simulink model "nonlinear_closed_backstepping_0"  (R2023b)
settings: Solver=ode45  StartTime=0.0  StopTime=100  FixedStep=0.001  MaxStep=1e-3  RelTol=1e-3  EnableMultiTasking=on
PreLoadFcn:
  | S=load('rovmodel75kg.mat'); M_nom=S.M; Ma_nom=S.Ma; DL_nom=S.DL; clear S;
values from neighbouring files (symbols this model uses):
  B = 735.75    [rovmodel75kg.mat]
  DL = [3.221 0 0 0 0 0 0 3.291 0 0 0 0 ... (36 elements, 6x6)]    [rovmodel75kg.mat]
  DQ = [105.3 0 0 0 0 0 0 139.6 0 0 0 0 ... (36 elements, 6x6)]    [rovmodel75kg.mat]
  I = [2.51  0  0; 0  3.38  0.01; 0  0.01  1.73]    [rovmodel75kg.mat]
  m = [75  0  0; 0  75  0; 0  0  75]    [rovmodel75kg.mat]
  M = [75 0 0 0 0 0 0 75 0 0 0 0 ... (36 elements, 6x6)]    [rovmodel75kg.mat]
  Ma = [-20.392 0 0 0 0 0 0 -53.435 0 0 0 0 ... (36 elements, 6x6)]    [rovmodel75kg.mat]
  rg = [0 0 0]    [rovmodel75kg.mat]
  W = 735.75    [rovmodel75kg.mat]
  zb = -0.397    [rovmodel75kg.mat]
  zg = 0    [rovmodel75kg.mat]
libraries: matrix_library x6
settings Model: Creator=Joshua cheng  LastModifiedBy=yhm
settings SolverCC: AlgebraicLoopSolver=TrustRegion
settings DataIOCC: LimitDataPoints=on  SaveFormat=Array  SignalLoggingSaveFormat=ModelDataLogs  ReturnWorkspaceOutputs=off
settings OptimizationCC: BlockReduction=off  OptimizeBlockIOStorage=off  BufferReuse=off  GlobalBufferReuse=off  ExpressionFolding=off  ExpressionDepthLimit=2147483647  LocalBlockOutputs=off  LifeSpan=inf  OptimizeDataStoreBuffers=off  BusAssignmentInplaceUpdate=off
settings DebuggingCC: SaveWithParameterizedLinksMsg=none  UnderspecifiedInitializationDetection=Classic  MergeDetectMultiDrivingBlocksExec=none  SolverPrmCheckMsg=warning  FcnCallInpInsideContextMsg=warning  UnconnectedInputMsg=warning  UnconnectedOutputMsg=warning  UnconnectedLineMsg=warning  StateNameClashWarn=warning  SFUnexpectedBacktrackingDiag=warning  SFNoUnconditionalDefaultTransitionDiag=warning  SFExecutionAtInitializationDiag=none  ArithmeticOperatorsInVariantConditions=warning
settings HardwareCC: ProdBitPerPointer=32  ProdBitPerSizeT=32  ProdBitPerPtrDiffT=32  ProdLargestAtomicFloat=None  ProdEndianess=BigEndian  ProdWordSize=32  ProdHWDeviceType=Specified  TargetIntDivRoundTo=Zero  TargetEndianess=BigEndian
settings ModelReferenceCC: EnableRefExpFcnMdlSchedulingChecks=on  PropagateSignalLabelsOutOfModel=off
settings SFSimCC: SimUseLocalCustomCode=off  CustomCodeUndefinedFunction=UseInterfaceOnly
settings RTWCC: Description=dSPACE DS1104 Hardware Platform  SystemTargetFile=rti1104.tlc  MakeCommand=make_rti  TemplateMakefile=rti1104.tmf  RTWUseLocalCustomCode=off  DLArmComputeVersion=19.05
settings CodeAppCC: StateflowObjectComments=on
settings STFCustomTargetCC: TargetLangStandard=C89/C90 (ANSI)  MatFileLogging=on  CPPClassGenCompliant=on  GRTInterface=on  SystemTargetFile=rti1104.tlc
settings GRTTargetCC: TargetLangStandard=C89/C90 (ANSI)  ParMdlRefBuildCompliant=off  CompOptLevelCompliant=off  ConcurrentExecutionCompliant=off  CombineOutputUpdateFcns=off  GRTInterface=on  UseToolchainInfoCompliant=off  ExtModeMexFile=noextcomm
settings ConfigComp: CovMetricSettings=dw  CovSaveCumulativeToWorkspaceVar=on  CovSaveSingleToWorkspaceVar=on  CovExternalEMLEnable=off

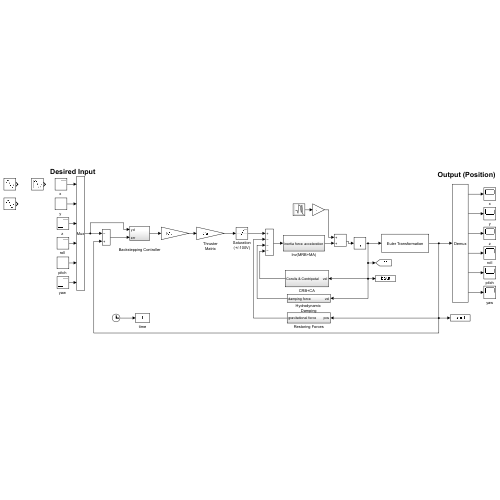
[thumbnail: Simulink's stored preview of the top-level diagram]
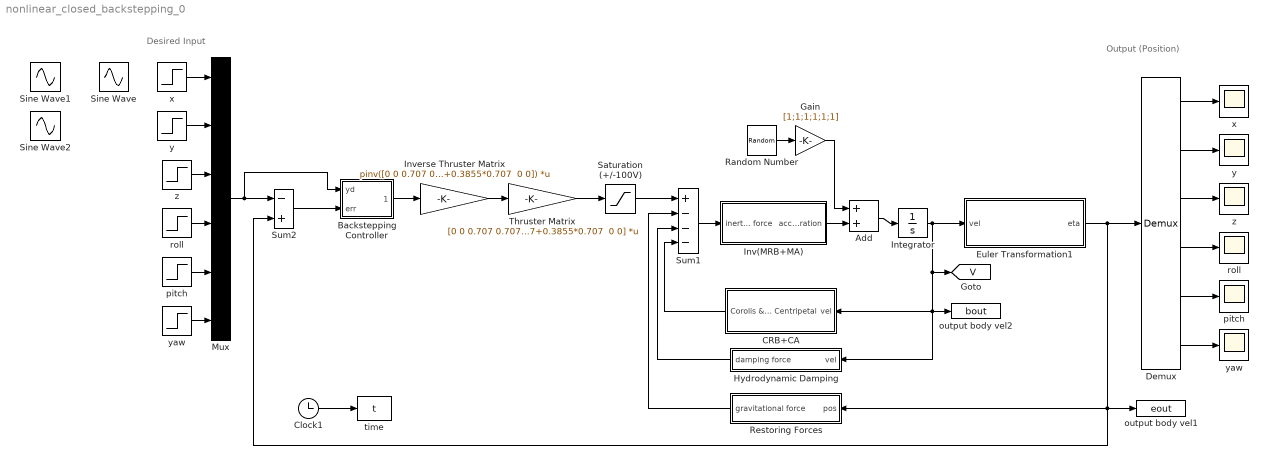
== system nonlinear_closed_backstepping_0 ==
  note: Desired Input
  note: Output (Position)
  " Backstepping Controller" : Subsystem
  Add : Sum
  CRB+CA : Subsystem
  Clock1 : Clock
  Demux : Demux  Outputs=6
      settings: DisplayOption=none
  Euler Transformation1 : Subsystem  AncestorBlock=rov_design_analysis/Scope Utilities/Euler Transformation
      mask Display: disp('Euler Transformation')
  Gain : Gain  Gain=[1;1;1;1;1;1]
  Hydrodynamic Damping : Subsystem
  Integrator : Integrator  InitialCondition=0.1
  Inv(MRB+MA) : Subsystem
  "Inverse Thruster Matrix " : Gain  Gain=|  Multiplication=Matrix(K*u)  SaturateOnIntegerOverflow=on  OutDataTypeStr=Inherit: Same as input  ParamDataTypeStr=Inherit: Same as input
      | pinv([0 0 0.707 0.707 0 0; 
      |     -0.707 0.707 0.707 -0.707 0 0; 
      |     0.707  0.707  0 0 1 1;
      |     -0.275*0.707+0.4305*0.707 0.275*0.707-0.4305*0.707  0  0  -0.275 0.275;
      |     0.3945*0.707 0.3945*0.707  0.4305*0.707  0.4305*0.707  -0.0355  -0.0355;
      |       -0.3945*0.707  0.3945*0.707  -0.275*0.707-0.3855*0.707  0.275*0.707+0.3855*0.707  0 0])
  Mux : Mux  Inputs=6
  Random Number : RandomNumber  Variance=0.001  SampleTime=0.1
  Restoring Forces : Subsystem
  Saturation (+/-100V) : Saturate  UpperLimit=100  LowerLimit=-100  ZeroCross=off
  Sine Wave : Sin  Frequency=0.1  SampleTime=0
  Sine Wave1 : Sin  Amplitude=2  Frequency=0.2  Phase=pi/2  SampleTime=0
  Sine Wave2 : Sin  Amplitude=2  Frequency=0.2  SampleTime=0
  Sum1 : Sum  Inputs=+---  InputSameDT=on  SaturateOnIntegerOverflow=on  OutDataTypeStr=Inherit: Same as first input
  Sum2 : Sum  Inputs=-+  InputSameDT=on  SaturateOnIntegerOverflow=on  OutDataTypeStr=Inherit: Same as first input
  "Thruster Matrix " : Gain  Gain=|  Multiplication=Matrix(K*u)  SaturateOnIntegerOverflow=on  OutDataTypeStr=Inherit: Same as input  ParamDataTypeStr=Inherit: Same as input
      | [0 0 0.707 0.707 0 0; 
      |     -0.707 0.707 0.707 -0.707 0 0; 
      |     0.707  0.707  0 0 1 1;
      |     -0.275*0.707+0.4305*0.707 0.275*0.707-0.4305*0.707  0  0  -0.275 0.275;
      |     0.3945*0.707 0.3945*0.707  0.4305*0.707  0.4305*0.707  -0.0355  -0.0355;
      |       -0.3945*0.707  0.3945*0.707  -0.275*0.707-0.3855*0.707  0.275*0.707+0.3855*0.707  0 0]
  output body vel1 : ToWorkspace  VariableName=eout  SampleTime=-1
  output body vel2 : ToWorkspace  VariableName=bout  SampleTime=-1
  pitch : Scope
  "pitch " : Step  Time=0  After=0  SampleTime=0
  roll : Scope
  "roll " : Step  Time=0  After=0  SampleTime=0
  time : ToWorkspace  VariableName=t  SampleTime=-1
  x : Scope
  "x " : Step  Time=0  After=2  SampleTime=0
  y : Scope
  "y " : Step  Time=0  After=2  SampleTime=0
  yaw : Scope
  "yaw " : Step  Time=0  After=0  SampleTime=0
  z : Scope
  "z " : Step  Time=0  After=2  SampleTime=0
  tag scope: V=global
  wires:
  Euler Transformation1/1("eta ") -> Demux/1, Sum2/2, output body vel1/1, Restoring Forces/1(pos)
  Integrator/1 -> Euler Transformation1/1(vel), CRB+CA/1(vel), Hydrodynamic Damping/1(vel), output body vel2/1, [V]
  Sum1/1 -> Inv(MRB+MA)/1(inertia force)
  "z "/1 -> Mux/3
  "roll "/1 -> Mux/4
  "pitch "/1 -> Mux/5
  Demux/6 -> yaw/1
  Demux/3 -> z/1
  Demux/4 -> roll/1
  Demux/5 -> pitch/1
  Demux/2 -> y/1
  Demux/1 -> x/1
  Mux/1 -> " Backstepping Controller"/1(yd), Sum2/1
  Sum2/1 -> " Backstepping Controller"/2(err)
  Saturation (+/-100V)/1 -> Sum1/1
  "yaw "/1 -> Mux/6
  " Backstepping Controller"/1(" ") -> "Inverse Thruster Matrix "/1
  "Inverse Thruster Matrix "/1 -> "Thruster Matrix "/1
  "Thruster Matrix "/1 -> Saturation (+/-100V)/1
  CRB+CA/1(Corolis & Centripetal) -> Sum1/4
  Hydrodynamic Damping/1(damping force) -> Sum1/3
  Restoring Forces/1(gravitational force) -> Sum1/2
  Clock1/1 -> time/1
  Random Number/1 -> Gain/1
  Gain/1 -> Add/1
  Inv(MRB+MA)/1(acceleration) -> Add/2
  Add/1 -> Integrator/1
  "x "/1 -> Mux/1
  "y "/1 -> Mux/2

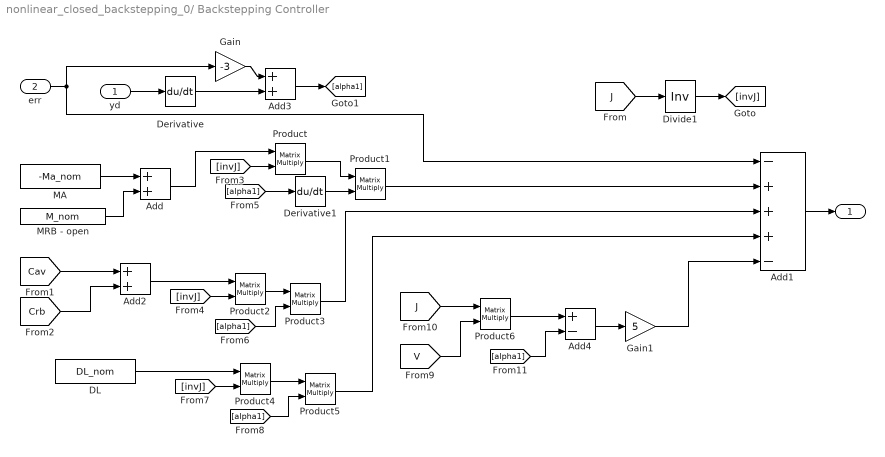
== system nonlinear_closed_backstepping_0/ Backstepping Controller ==
  yd : Inport
  err : Inport  Port=2
  Add : Sum
  Add1 : Sum  Inputs=-+++-
  Add2 : Sum
  Add3 : Sum
  Add4 : Sum  Inputs=+-
  DL : Constant  Value=DL_nom
  Derivative : Derivative
  Derivative1 : Derivative
  Divide1 : Product  Inputs=/  Multiplication=Matrix(*)
  Gain : Gain  Gain=-3
  Gain1 : Gain  Gain=5
  MA : Constant  Value=-Ma_nom
  MRB - open : Constant  Value=M_nom
  Product{,1..6} (7 alike) : Product  Multiplication=Matrix(*)
  " " : Outport
  wires:
  err/1 -> Add1/1, Gain/1
  MA/1 -> Add/1
  MRB - open/1 -> Add/2
  [J] -> Divide1/1
  Add/1 -> Product/1
  yd/1 -> Derivative/1
  Product/1 -> Product1/1
  [Crb] -> Add2/2
  [Cav] -> Add2/1
  Divide1/1 -> [invJ]
  [invJ] -> Product/2
  Add2/1 -> Product2/1
  [invJ] -> Product2/2
  Product2/1 -> Product3/1
  Derivative/1 -> Add3/2
  Gain/1 -> Add3/1
  Add3/1 -> [alpha1]
  [alpha1] -> Product3/2
  Derivative1/1 -> Product1/2
  [alpha1] -> Derivative1/1
  DL/1 -> Product4/1
  [invJ] -> Product4/2
  Product4/1 -> Product5/1
  [alpha1] -> Product5/2
  [J] -> Product6/1
  [V] -> Product6/2
  Product6/1 -> Add4/1
  [alpha1] -> Add4/2
  Add4/1 -> Gain1/1
  Gain1/1 -> Add1/5
  Add1/1 -> " "/1
  Product5/1 -> Add1/4
  Product3/1 -> Add1/3
  Product1/1 -> Add1/2

== system nonlinear_closed_backstepping_0/CRB+CA ==
  vel : Inport
  Add2 : Sum
  Centripetal & Coriolis : Subsystem  AncestorBlock=rov_design_analysis/ROV Models/1. Six DOF RRC ROV II/Centripetal & Coriolis
      mask Display: disp('CRB')
  Centripetal & Coriolis1 : Subsystem  AncestorBlock=rov_design_analysis/ROV Models/1. Six DOF RRC ROV II/Centripetal & Coriolis
      mask Display: disp('CA')
  Product5 : Product  Multiplication=Matrix(*)
  Subsystem : Subsystem
      mask Display: disp('CRB(v)')
  Corolis & Centripetal : Outport
  tag scope: Cav=global, Crb=global
  wires:
  Add2/1 -> Product5/1
  vel/1 -> Product5/2, Subsystem/1(In1), Centripetal & Coriolis1/1(vel)
  Product5/1 -> Corolis & Centripetal/1
  Subsystem/1(Out1) -> Add2/2, [Crb]
  Centripetal & Coriolis1/1(Ca) -> [Cav], Add2/1

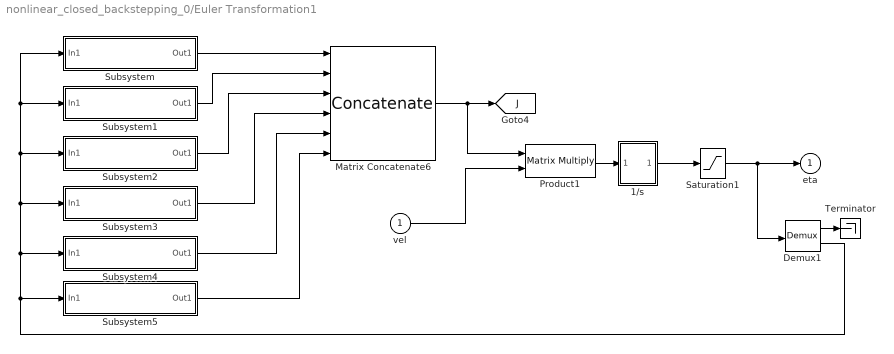
== system nonlinear_closed_backstepping_0/Euler Transformation1 ==
  vel : Inport
  1/s : Subsystem
  Demux1 : Demux  Outputs=2
      settings: DisplayOption=none
  Matrix Concatenate6 : Concatenate  NumInputs=6  Mode=Multidimensional array
  Product1 : Product  Multiplication=Matrix(*)  RndMeth=Zero
  Saturation1 : Saturate  UpperLimit=360  LowerLimit=-360
  Subsystem : Subsystem
      mask Display: disp('Transformation J first Row')
  Subsystem1 : Subsystem
      mask Display: disp('Transformation J second Row')
  Subsystem2 : Subsystem
      mask Display: disp('Transformation J third Row')
  Subsystem3 : Subsystem
      mask Display: disp('Transformation J fourth Row')
  Subsystem4 : Subsystem
      mask Display: disp('Transformation J fifth Row')
  Subsystem5 : Subsystem
      mask Display: disp('Transformation J sixth Row')
  Terminator : Terminator
  "eta " : Outport  InitialOutput=0
  tag scope: J=global
  wires:
  vel/1 -> Product1/2
  Demux1/1 -> Terminator/1
  Saturation1/1 -> "eta "/1, Demux1/1
  Matrix Concatenate6/1 -> Product1/1, [J]
  Subsystem/1(Out1) -> Matrix Concatenate6/1
  Demux1/2 -> Subsystem/1(In1), Subsystem1/1(In1), Subsystem2/1(In1), Subsystem3/1(In1), Subsystem4/1(In1), Subsystem5/1(In1)
  Subsystem1/1(Out1) -> Matrix Concatenate6/2
  Subsystem2/1(Out1) -> Matrix Concatenate6/3
  Subsystem3/1(Out1) -> Matrix Concatenate6/4
  Subsystem4/1(Out1) -> Matrix Concatenate6/5
  Subsystem5/1(Out1) -> Matrix Concatenate6/6
  1/s/1(Out1) -> Saturation1/1
  Product1/1 -> 1/s/1(In1)

== system nonlinear_closed_backstepping_0/Hydrodynamic Damping ==
  vel : Inport
  Abs : Abs  SaturateOnIntegerOverflow=off
  Add : Sum
  Constant : Constant  Value=0
  D linear : Gain  Gain=diag(DL)  SaturateOnIntegerOverflow=on  OutDataTypeStr=Inherit: Same as input  ParamDataTypeStr=Inherit: Same as input
  D quadratic : Gain  Gain=diag(DQ)  SaturateOnIntegerOverflow=on  OutDataTypeStr=Inherit: Same as input  ParamDataTypeStr=Inherit: Same as input
  Manual Switch : ManualSwitch
  Manual Switch1 : ManualSwitch
  Product : Product  RndMeth=Zero
  damping force : Outport  InitialOutput=0
  wires:
  vel/1 -> D linear/1, Abs/1, Product/2
  D linear/1 -> Manual Switch/1
  Add/1 -> damping force/1
  Abs/1 -> D quadratic/1
  D quadratic/1 -> Product/1
  Manual Switch/1 -> Add/1
  Product/1 -> Manual Switch/2, Manual Switch1/2
  Manual Switch1/1 -> Add/2
  Constant/1 -> Manual Switch1/1

== system nonlinear_closed_backstepping_0/Inv(MRB+MA) ==
  note: TauA-Cv-Dv-Gf
  inertia force : Inport
  Divide : Product  Inputs=/  Multiplication=Matrix(*)
  MA : Constant  Value=-Ma
  "MRB " : Constant  Value=M
  Product : Product  Multiplication=Matrix(*)  RndMeth=Zero
  Sum1 : Sum  InputSameDT=on  SaturateOnIntegerOverflow=on  OutDataTypeStr=Inherit: Same as first input
  acceleration : Outport
  wires:
  Divide/1 -> Product/1
  Product/1 -> acceleration/1
  inertia force/1 -> Product/2
  MA/1 -> Sum1/2
  Sum1/1 -> Divide/1
  "MRB "/1 -> Sum1/1

== system nonlinear_closed_backstepping_0/Restoring Forces ==
  pos : Inport
  (zg.W - zb.B)cY.sX : Fcn  Expr=((zg * W - zb * B) * cos(u[2])) * sin(u[1])
  (zg.W - zb.B)sY : Fcn  Expr=(zg*W - zb*B)*sin(u[2])
  -(xg.W-xb.B)cY.sX : Fcn  Expr=0
  -cY.cX : Fcn  Expr=0
  -cY.sX : Fcn  Expr=0
  Demux : Demux  Outputs=2
      settings: DisplayOption=none
  Mux1 : Mux  Inputs=6
  Terminator : Terminator
  sY : Fcn  Expr=0
  gravitational force : Outport  InitialOutput=0
  wires:
  Mux1/1 -> gravitational force/1
  Demux/2 -> (zg.W - zb.B)cY.sX/1, -(xg.W-xb.B)cY.sX/1, (zg.W - zb.B)sY/1, sY/1, -cY.sX/1, -cY.cX/1  "pos_2"
  Demux/1 -> Terminator/1  "pos_1"
  pos/1 -> Demux/1
  sY/1 -> Mux1/1
  -cY.sX/1 -> Mux1/2
  -cY.cX/1 -> Mux1/3
  (zg.W - zb.B)cY.sX/1 -> Mux1/4
  (zg.W - zb.B)sY/1 -> Mux1/5
  -(xg.W-xb.B)cY.sX/1 -> Mux1/6

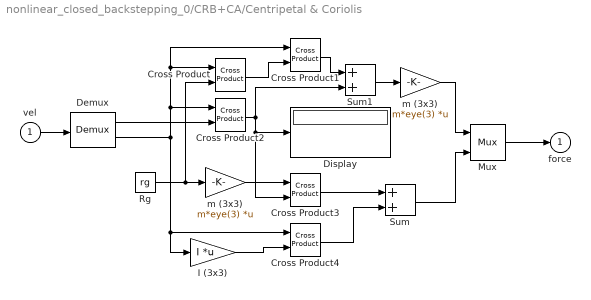
== system nonlinear_closed_backstepping_0/CRB+CA/Centripetal & Coriolis ==
  vel : Inport
  Cross Product{,1..4} (5 alike) : matrix_library/Cross Product
  Demux : Demux  Outputs=2
      settings: DisplayOption=none
  Display : Display
  "I (3x3) " : Gain  Gain=I  Multiplication=Matrix(K*u)  SaturateOnIntegerOverflow=on  OutDataTypeStr=Inherit: Same as input  ParamDataTypeStr=Inherit: Same as input
  Mux : Mux  Inputs=2
  Rg : Constant  Value=rg
  Sum : Sum  InputSameDT=on  SaturateOnIntegerOverflow=on  OutDataTypeStr=Inherit: Same as first input
  Sum1 : Sum  InputSameDT=on  SaturateOnIntegerOverflow=on  OutDataTypeStr=Inherit: Same as first input
  m (3x3) : Gain  Gain=m*eye(3)  Multiplication=Matrix(K*u)  SaturateOnIntegerOverflow=on  OutDataTypeStr=Inherit: Same as input  ParamDataTypeStr=Inherit: Same as input
  "m (3x3) " : Gain  Gain=m*eye(3)  Multiplication=Matrix(K*u)  SaturateOnIntegerOverflow=on  OutDataTypeStr=Inherit: Same as input  ParamDataTypeStr=Inherit: Same as input
  force : Outport  InitialOutput=0
  wires:
  Cross Product4/1 -> Sum/2
  "m (3x3) "/1 -> Cross Product3/1
  Cross Product3/1 -> Sum/1
  Cross Product/1 -> Cross Product1/2
  Cross Product1/1 -> Sum1/1
  Sum1/1 -> m (3x3)/1
  vel/1 -> Demux/1
  m (3x3)/1 -> Mux/1
  Sum/1 -> Mux/2
  Mux/1 -> force/1
  Demux/2 -> Cross Product2/1, Cross Product1/1, Cross Product/1, Cross Product4/1, "I (3x3) "/1
  Rg/1 -> Cross Product/2, "m (3x3) "/1
  "I (3x3) "/1 -> Cross Product4/2
  Cross Product2/1 -> Cross Product3/2, Display/1, Sum1/2
  Demux/1 -> Cross Product2/2

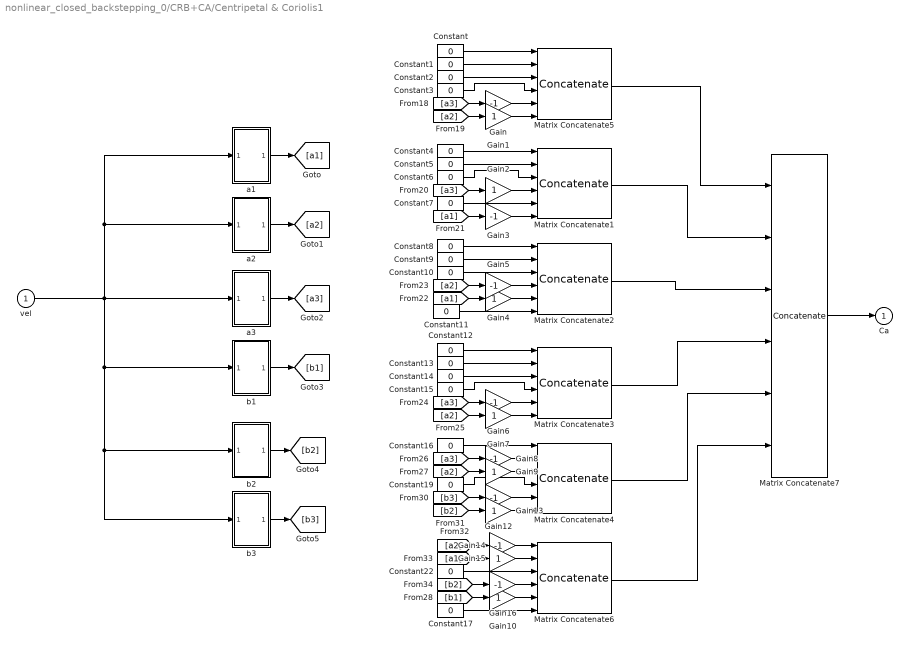
== system nonlinear_closed_backstepping_0/CRB+CA/Centripetal & Coriolis1 ==
  vel : Inport
  Constant{,1..17,19,22} (20 alike) : Constant  Value=0
  Gain{,3,5..6,8,12,14,16} (8 alike) : Gain  Gain=-1
  Gain{1..2,4,7,9..10,13,15} (8 alike) : Gain
  Matrix Concatenate{1..6} (6 alike) : Concatenate  NumInputs=6  Mode=Multidimensional array  ConcatenateDimension=2
  Matrix Concatenate7 : Concatenate  NumInputs=6  Mode=Multidimensional array
  a1 : Subsystem
      mask Display: disp('Row 1')
  a2 : Subsystem
      mask Display: disp('Row 2')
  a3 : Subsystem
      mask Display: disp('Row 1')
  b1 : Subsystem
      mask Display: disp('Row 2')
  b2 : Subsystem
      mask Display: disp('Row 1')
  b3 : Subsystem
      mask Display: disp('Row 2')
  Ca : Outport  InitialOutput=0
  wires:
  vel/1 -> b3/1(In1), b2/1(In1), b1/1(In1), a3/1(In1), a1/1(In1), a2/1(In1)
  a1/1(Out1) -> [a1]
  b2/1(Out1) -> [b2]
  a3/1(Out1) -> [a3]
  a2/1(Out1) -> [a2]
  b1/1(Out1) -> [b1]
  b3/1(Out1) -> [b3]
  Constant/1 -> Matrix Concatenate5/1
  Gain/1 -> Matrix Concatenate5/5
  Gain1/1 -> Matrix Concatenate5/6
  Constant1/1 -> Matrix Concatenate5/2
  Constant2/1 -> Matrix Concatenate5/3
  Constant3/1 -> Matrix Concatenate5/4
  [a3] -> Gain/1
  [a2] -> Gain1/1
  Constant5/1 -> Matrix Concatenate1/2
  [a3] -> Gain2/1
  [a1] -> Gain3/1
  Gain3/1 -> Matrix Concatenate1/6
  Constant4/1 -> Matrix Concatenate1/1
  Constant10/1 -> Matrix Concatenate2/3
  Constant9/1 -> Matrix Concatenate2/2
  [a1] -> Gain4/1
  [a2] -> Gain5/1
  Gain4/1 -> Matrix Concatenate2/5
  Constant8/1 -> Matrix Concatenate2/1
  Constant14/1 -> Matrix Concatenate3/3
  Constant13/1 -> Matrix Concatenate3/2
  [a3] -> Gain6/1
  Constant15/1 -> Matrix Concatenate3/4
  [a2] -> Gain7/1
  Gain7/1 -> Matrix Concatenate3/6
  Gain6/1 -> Matrix Concatenate3/5
  Constant12/1 -> Matrix Concatenate3/1
  Gain8/1 -> Matrix Concatenate4/2
  [a3] -> Gain8/1
  Constant19/1 -> Matrix Concatenate4/4
  [a2] -> Gain9/1
  Constant16/1 -> Matrix Concatenate4/1
  Constant22/1 -> Matrix Concatenate6/3
  [b1] -> Gain10/1
  Gain10/1 -> Matrix Concatenate6/5
  Gain2/1 -> Matrix Concatenate1/4
  Constant6/1 -> Matrix Concatenate1/3
  Constant7/1 -> Matrix Concatenate1/5
  Gain5/1 -> Matrix Concatenate2/4
  Constant11/1 -> Matrix Concatenate2/6
  Gain9/1 -> Matrix Concatenate4/3
  [b3] -> Gain12/1
  Gain12/1 -> Matrix Concatenate4/5
  Gain13/1 -> Matrix Concatenate4/6
  [b2] -> Gain13/1
  Gain14/1 -> Matrix Concatenate6/1
  [a2] -> Gain14/1
  Gain15/1 -> Matrix Concatenate6/2
  [a1] -> Gain15/1
  Gain16/1 -> Matrix Concatenate6/4
  [b2] -> Gain16/1
  Constant17/1 -> Matrix Concatenate6/6
  Matrix Concatenate5/1 -> Matrix Concatenate7/1
  Matrix Concatenate1/1 -> Matrix Concatenate7/2
  Matrix Concatenate2/1 -> Matrix Concatenate7/3
  Matrix Concatenate3/1 -> Matrix Concatenate7/4
  Matrix Concatenate4/1 -> Matrix Concatenate7/5
  Matrix Concatenate6/1 -> Matrix Concatenate7/6
  Matrix Concatenate7/1 -> Ca/1

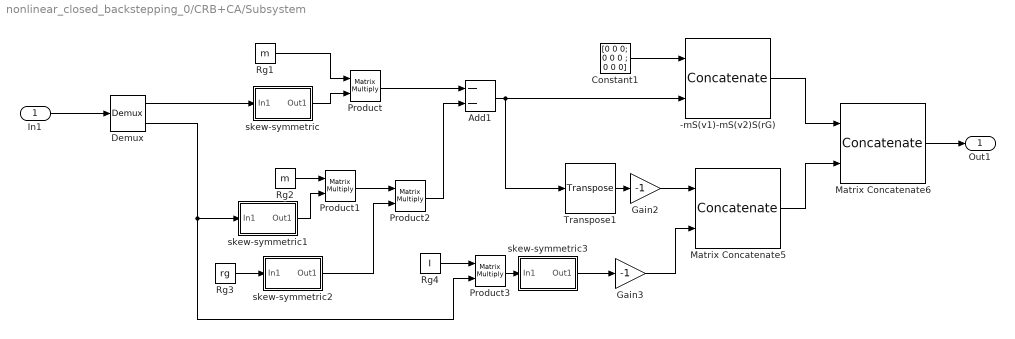
== system nonlinear_closed_backstepping_0/CRB+CA/Subsystem ==
  In1 : Inport
  -mS(v1)-mS(v2)S(rG) : Concatenate  Mode=Multidimensional array  ConcatenateDimension=2
  Add1 : Sum  Inputs=--
  Constant1 : Constant  Value=[0 0 0; 0 0 0 ; 0 0 0]
  Demux : Demux  Outputs=2
      settings: DisplayOption=none
  Gain2 : Gain  Gain=-1
  Gain3 : Gain  Gain=-1
  Matrix Concatenate5 : Concatenate  Mode=Multidimensional array  ConcatenateDimension=2
  Matrix Concatenate6 : Concatenate  Mode=Multidimensional array
  Product{,1..3} (4 alike) : Product  Multiplication=Matrix(*)
  Rg1 : Constant  Value=m
  Rg2 : Constant  Value=m
  Rg3 : Constant  Value=rg
  Rg4 : Constant  Value=I
  Transpose1 : matrix_library/Transpose
  skew-symmetric : Subsystem
  skew-symmetric1 : Subsystem
  skew-symmetric2 : Subsystem
  skew-symmetric3 : Subsystem
  Out1 : Outport
  wires:
  In1/1 -> Demux/1
  Rg2/1 -> Product1/1
  Product3/1 -> skew-symmetric3/1(In1)
  skew-symmetric1/1(Out1) -> Product1/2
  Rg3/1 -> skew-symmetric2/1(In1)
  Matrix Concatenate5/1 -> Matrix Concatenate6/2
  Rg4/1 -> Product3/1
  Constant1/1 -> -mS(v1)-mS(v2)S(rG)/1
  Demux/2 -> Product3/2, skew-symmetric1/1(In1)
  Gain3/1 -> Matrix Concatenate5/2
  Add1/1 -> -mS(v1)-mS(v2)S(rG)/2, Transpose1/1
  Product2/1 -> Add1/2
  Gain2/1 -> Matrix Concatenate5/1
  Matrix Concatenate6/1 -> Out1/1
  skew-symmetric3/1(Out1) -> Gain3/1
  Transpose1/1 -> Gain2/1
  skew-symmetric2/1(Out1) -> Product2/2
  skew-symmetric/1(Out1) -> Product/2
  Demux/1 -> skew-symmetric/1(In1)
  -mS(v1)-mS(v2)S(rG)/1 -> Matrix Concatenate6/1
  Rg1/1 -> Product/1
  Product/1 -> Add1/1
  Product1/1 -> Product2/1

== system nonlinear_closed_backstepping_0/Euler Transformation1/1//s ==
  In1 : Inport
  Demux2 : Demux  Outputs=6
      settings: DisplayOption=none
  Integrator{,1..2,4..6} (6 alike) : Integrator
  Mux2 : Mux  Inputs=6
  Out1 : Outport
  wires:
  Demux2/1 -> Integrator/1
  Demux2/2 -> Integrator1/1
  Demux2/3 -> Integrator2/1
  Demux2/4 -> Integrator4/1
  Demux2/5 -> Integrator5/1
  Integrator/1 -> Mux2/1
  Integrator1/1 -> Mux2/2
  Integrator2/1 -> Mux2/3
  Integrator4/1 -> Mux2/4
  In1/1 -> Demux2/1
  Mux2/1 -> Out1/1
  Integrator5/1 -> Mux2/5
  Demux2/6 -> Integrator6/1
  Integrator6/1 -> Mux2/6

== system nonlinear_closed_backstepping_0/Euler Transformation1/Subsystem ==
  In1 : Inport
  -sZ.cX+cZ.sY.sX : Fcn  Expr=-sin(u[3])*cos(u[1]) + cos(u[3])*sin(u[2])*sin(u[1])
  Constant : Constant  Value=0
  Matrix Concatenate : Concatenate  NumInputs=6  Mode=Multidimensional array  ConcatenateDimension=2
  cY.cZ : Fcn  Expr=cos(u[3]) * cos(u[2])
  sZ.sX+cZ.cX.sY : Fcn  Expr=sin(u[3])*sin(u[1]) + cos(u[3])*cos(u[1])*sin(u[2])
  Out1 : Outport
  wires:
  Constant/1 -> Matrix Concatenate/6, Matrix Concatenate/5, Matrix Concatenate/4
  cY.cZ/1 -> Matrix Concatenate/1
  Matrix Concatenate/1 -> Out1/1
  sZ.sX+cZ.cX.sY/1 -> Matrix Concatenate/3
  -sZ.cX+cZ.sY.sX/1 -> Matrix Concatenate/2
  In1/1 -> sZ.sX+cZ.cX.sY/1, -sZ.cX+cZ.sY.sX/1, cY.cZ/1

== system nonlinear_closed_backstepping_0/Euler Transformation1/Subsystem1 ==
  In1 : Inport
  -cZ.sX+sY.sZ.cX : Fcn  Expr=-cos(u[3])*sin(u[1]) + sin(u[2])*sin(u[3])*cos(u[1])
  Constant1 : Constant  Value=0
  Matrix Concatenate1 : Concatenate  NumInputs=6  Mode=Multidimensional array  ConcatenateDimension=2
  cY.sZ : Fcn  Expr=sin(u[3]) * cos(u[2])
  cZ.cX+sX.sY.sZ : Fcn  Expr=cos(u[3])*cos(u[1]) + sin(u[1])*sin(u[2])*sin(u[3])
  Out1 : Outport
  wires:
  cY.sZ/1 -> Matrix Concatenate1/1
  Matrix Concatenate1/1 -> Out1/1
  -cZ.sX+sY.sZ.cX/1 -> Matrix Concatenate1/3
  cZ.cX+sX.sY.sZ/1 -> Matrix Concatenate1/2
  Constant1/1 -> Matrix Concatenate1/6, Matrix Concatenate1/5, Matrix Concatenate1/4
  In1/1 -> -cZ.sX+sY.sZ.cX/1, cZ.cX+sX.sY.sZ/1, cY.sZ/1

== system nonlinear_closed_backstepping_0/Euler Transformation1/Subsystem2 ==
  In1 : Inport
  -sY : Fcn  Expr=-sin(u[2])
  Constant2 : Constant  Value=0
  Matrix Concatenate2 : Concatenate  NumInputs=6  Mode=Multidimensional array  ConcatenateDimension=2
  cY.cX : Fcn  Expr=cos(u[2])*cos(u[1])
  cY.sX : Fcn  Expr=cos(u[2])*sin(u[1])
  Out1 : Outport
  wires:
  Matrix Concatenate2/1 -> Out1/1
  Constant2/1 -> Matrix Concatenate2/6, Matrix Concatenate2/5, Matrix Concatenate2/4
  cY.sX/1 -> Matrix Concatenate2/2
  cY.cX/1 -> Matrix Concatenate2/3
  -sY/1 -> Matrix Concatenate2/1
  In1/1 -> cY.cX/1, cY.sX/1, -sY/1

== system nonlinear_closed_backstepping_0/Euler Transformation1/Subsystem3 ==
  In1 : Inport
  1 : Fcn  Expr=1
  Constant3 : Constant  Value=0
  Matrix Concatenate3 : Concatenate  NumInputs=6  Mode=Multidimensional array  ConcatenateDimension=2
  cX.tY : Fcn  Expr=cos(u[1])*tan(u[2])
  sX.tY : Fcn  Expr=sin(u[1])*tan(u[2])
  Out1 : Outport
  wires:
  cX.tY/1 -> Matrix Concatenate3/6
  sX.tY/1 -> Matrix Concatenate3/5
  1/1 -> Matrix Concatenate3/4
  Constant3/1 -> Matrix Concatenate3/3, Matrix Concatenate3/2, Matrix Concatenate3/1
  Matrix Concatenate3/1 -> Out1/1
  In1/1 -> cX.tY/1, sX.tY/1, 1/1

== system nonlinear_closed_backstepping_0/Euler Transformation1/Subsystem4 ==
  In1 : Inport
  -sX : Fcn  Expr=-sin(u[1])
  0 : Fcn  Expr=0
  Constant4 : Constant  Value=0
  Dot Product1 : Subsystem
  Matrix Concatenate4 : Concatenate  NumInputs=6  Mode=Multidimensional array  ConcatenateDimension=2
  cX : Fcn  Expr=cos(u[1])
  Out1 : Outport
  wires:
  In1/1 -> -sX/1, cX/1, 0/1
  cX/1 -> Matrix Concatenate4/5
  0/1 -> Matrix Concatenate4/4
  Matrix Concatenate4/1 -> Out1/1
  Constant4/1 -> Matrix Concatenate4/3, Matrix Concatenate4/2, Matrix Concatenate4/1
  -sX/1 -> Matrix Concatenate4/6

== system nonlinear_closed_backstepping_0/Euler Transformation1/Subsystem5 ==
  In1 : Inport
  2 : Fcn  Expr=0
  Constant5 : Constant  Value=0
  Matrix Concatenate5 : Concatenate  NumInputs=6  Mode=Multidimensional array  ConcatenateDimension=2
  cX/cY : Fcn  Expr=cos(u[1])/cos(u[2])
  sX/cY : Fcn  Expr=sin(u[1])/cos(u[2])
  Out1 : Outport
  wires:
  Constant5/1 -> Matrix Concatenate5/3, Matrix Concatenate5/2, Matrix Concatenate5/1
  cX/cY/1 -> Matrix Concatenate5/6
  In1/1 -> cX/cY/1, sX/cY/1, 2/1
  2/1 -> Matrix Concatenate5/4
  sX/cY/1 -> Matrix Concatenate5/5
  Matrix Concatenate5/1 -> Out1/1

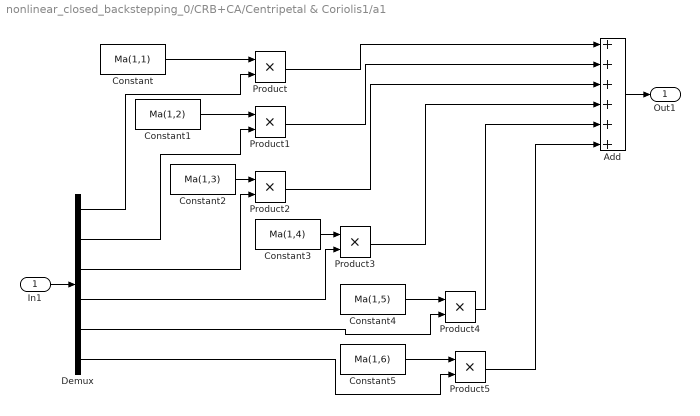
== system nonlinear_closed_backstepping_0/CRB+CA/Centripetal & Coriolis1/a1 ==
  In1 : Inport
  Add : Sum  Inputs=++++++
  Constant : Constant  Value=Ma(1,1)
  Constant1 : Constant  Value=Ma(1,2)
  Constant2 : Constant  Value=Ma(1,3)
  Constant3 : Constant  Value=Ma(1,4)
  Constant4 : Constant  Value=Ma(1,5)
  Constant5 : Constant  Value=Ma(1,6)
  Demux : Demux  Outputs=6
  Product{,1..5} (6 alike) : Product  RndMeth=Zero
  Out1 : Outport
  wires:
  Demux/1 -> Product/2
  Demux/2 -> Product1/2
  Demux/3 -> Product2/2
  Demux/4 -> Product3/2
  Demux/5 -> Product4/2
  Demux/6 -> Product5/2
  Product5/1 -> Add/6
  Constant5/1 -> Product5/1
  Product4/1 -> Add/5
  Constant4/1 -> Product4/1
  Product3/1 -> Add/4
  Constant3/1 -> Product3/1
  Product2/1 -> Add/3
  Constant2/1 -> Product2/1
  Product1/1 -> Add/2
  Constant1/1 -> Product1/1
  Product/1 -> Add/1
  Constant/1 -> Product/1
  Add/1 -> Out1/1
  In1/1 -> Demux/1

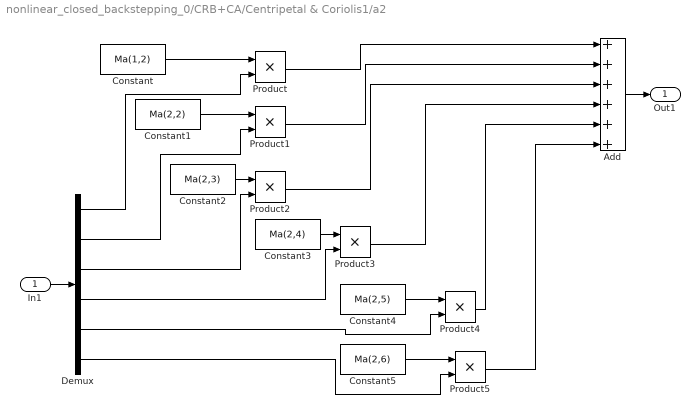
== system nonlinear_closed_backstepping_0/CRB+CA/Centripetal & Coriolis1/a2 ==
  In1 : Inport
  Add : Sum  Inputs=++++++
  Constant : Constant  Value=Ma(1,2)
  Constant1 : Constant  Value=Ma(2,2)
  Constant2 : Constant  Value=Ma(2,3)
  Constant3 : Constant  Value=Ma(2,4)
  Constant4 : Constant  Value=Ma(2,5)
  Constant5 : Constant  Value=Ma(2,6)
  Demux : Demux  Outputs=6
  Product{,1..5} (6 alike) : Product  RndMeth=Zero
  Out1 : Outport
  wires:
  Demux/1 -> Product/2
  Demux/2 -> Product1/2
  Demux/3 -> Product2/2
  Demux/4 -> Product3/2
  Demux/5 -> Product4/2
  Demux/6 -> Product5/2
  Product5/1 -> Add/6
  Constant5/1 -> Product5/1
  Product4/1 -> Add/5
  Constant4/1 -> Product4/1
  Product3/1 -> Add/4
  Constant3/1 -> Product3/1
  Product2/1 -> Add/3
  Constant2/1 -> Product2/1
  Product1/1 -> Add/2
  Constant1/1 -> Product1/1
  Product/1 -> Add/1
  Constant/1 -> Product/1
  Add/1 -> Out1/1
  In1/1 -> Demux/1

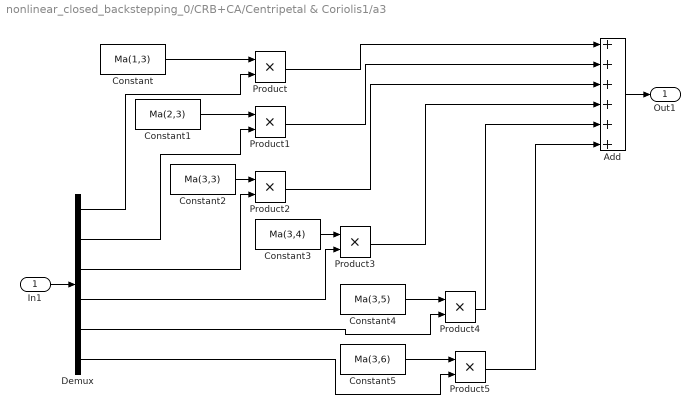
== system nonlinear_closed_backstepping_0/CRB+CA/Centripetal & Coriolis1/a3 ==
  In1 : Inport
  Add : Sum  Inputs=++++++
  Constant : Constant  Value=Ma(1,3)
  Constant1 : Constant  Value=Ma(2,3)
  Constant2 : Constant  Value=Ma(3,3)
  Constant3 : Constant  Value=Ma(3,4)
  Constant4 : Constant  Value=Ma(3,5)
  Constant5 : Constant  Value=Ma(3,6)
  Demux : Demux  Outputs=6
  Product{,1..5} (6 alike) : Product  RndMeth=Zero
  Out1 : Outport
  wires:
  Demux/1 -> Product/2
  Demux/2 -> Product1/2
  Demux/3 -> Product2/2
  Demux/4 -> Product3/2
  Demux/5 -> Product4/2
  Demux/6 -> Product5/2
  Product5/1 -> Add/6
  Constant5/1 -> Product5/1
  Product4/1 -> Add/5
  Constant4/1 -> Product4/1
  Product3/1 -> Add/4
  Constant3/1 -> Product3/1
  Product2/1 -> Add/3
  Constant2/1 -> Product2/1
  Product1/1 -> Add/2
  Constant1/1 -> Product1/1
  Product/1 -> Add/1
  Constant/1 -> Product/1
  Add/1 -> Out1/1
  In1/1 -> Demux/1

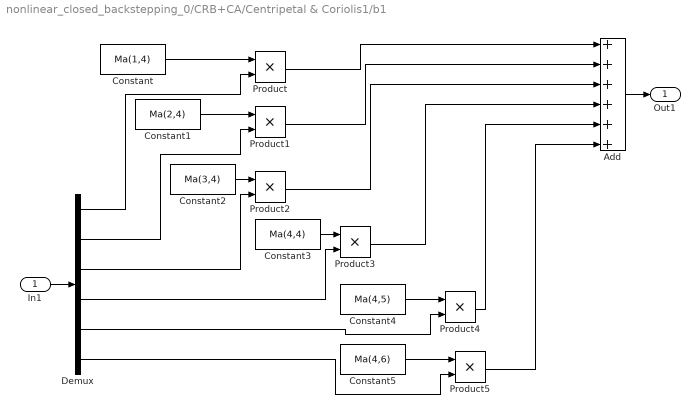
== system nonlinear_closed_backstepping_0/CRB+CA/Centripetal & Coriolis1/b1 ==
  In1 : Inport
  Add : Sum  Inputs=++++++
  Constant : Constant  Value=Ma(1,4)
  Constant1 : Constant  Value=Ma(2,4)
  Constant2 : Constant  Value=Ma(3,4)
  Constant3 : Constant  Value=Ma(4,4)
  Constant4 : Constant  Value=Ma(4,5)
  Constant5 : Constant  Value=Ma(4,6)
  Demux : Demux  Outputs=6
  Product{,1..5} (6 alike) : Product  RndMeth=Zero
  Out1 : Outport
  wires:
  Demux/1 -> Product/2
  Demux/2 -> Product1/2
  Demux/3 -> Product2/2
  Demux/4 -> Product3/2
  Demux/5 -> Product4/2
  Demux/6 -> Product5/2
  Product5/1 -> Add/6
  Constant5/1 -> Product5/1
  Product4/1 -> Add/5
  Constant4/1 -> Product4/1
  Product3/1 -> Add/4
  Constant3/1 -> Product3/1
  Product2/1 -> Add/3
  Constant2/1 -> Product2/1
  Product1/1 -> Add/2
  Constant1/1 -> Product1/1
  Product/1 -> Add/1
  Constant/1 -> Product/1
  Add/1 -> Out1/1
  In1/1 -> Demux/1

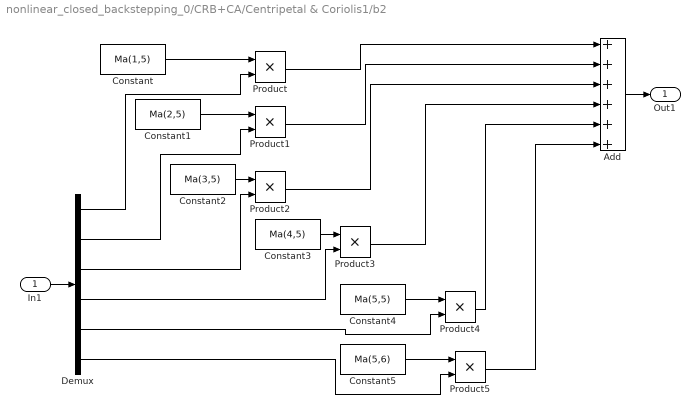
== system nonlinear_closed_backstepping_0/CRB+CA/Centripetal & Coriolis1/b2 ==
  In1 : Inport
  Add : Sum  Inputs=++++++
  Constant : Constant  Value=Ma(1,5)
  Constant1 : Constant  Value=Ma(2,5)
  Constant2 : Constant  Value=Ma(3,5)
  Constant3 : Constant  Value=Ma(4,5)
  Constant4 : Constant  Value=Ma(5,5)
  Constant5 : Constant  Value=Ma(5,6)
  Demux : Demux  Outputs=6
  Product{,1..5} (6 alike) : Product  RndMeth=Zero
  Out1 : Outport
  wires:
  Demux/1 -> Product/2
  Demux/2 -> Product1/2
  Demux/3 -> Product2/2
  Demux/4 -> Product3/2
  Demux/5 -> Product4/2
  Demux/6 -> Product5/2
  Product5/1 -> Add/6
  Constant5/1 -> Product5/1
  Product4/1 -> Add/5
  Constant4/1 -> Product4/1
  Product3/1 -> Add/4
  Constant3/1 -> Product3/1
  Product2/1 -> Add/3
  Constant2/1 -> Product2/1
  Product1/1 -> Add/2
  Constant1/1 -> Product1/1
  Product/1 -> Add/1
  Constant/1 -> Product/1
  Add/1 -> Out1/1
  In1/1 -> Demux/1

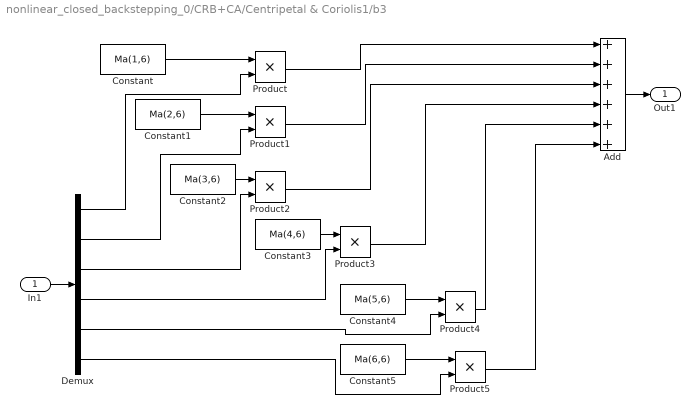
== system nonlinear_closed_backstepping_0/CRB+CA/Centripetal & Coriolis1/b3 ==
  In1 : Inport
  Add : Sum  Inputs=++++++
  Constant : Constant  Value=Ma(1,6)
  Constant1 : Constant  Value=Ma(2,6)
  Constant2 : Constant  Value=Ma(3,6)
  Constant3 : Constant  Value=Ma(4,6)
  Constant4 : Constant  Value=Ma(5,6)
  Constant5 : Constant  Value=Ma(6,6)
  Demux : Demux  Outputs=6
  Product{,1..5} (6 alike) : Product  RndMeth=Zero
  Out1 : Outport
  wires:
  Demux/1 -> Product/2
  Demux/2 -> Product1/2
  Demux/3 -> Product2/2
  Demux/4 -> Product3/2
  Demux/5 -> Product4/2
  Demux/6 -> Product5/2
  Product5/1 -> Add/6
  Constant5/1 -> Product5/1
  Product4/1 -> Add/5
  Constant4/1 -> Product4/1
  Product3/1 -> Add/4
  Constant3/1 -> Product3/1
  Product2/1 -> Add/3
  Constant2/1 -> Product2/1
  Product1/1 -> Add/2
  Constant1/1 -> Product1/1
  Product/1 -> Add/1
  Constant/1 -> Product/1
  Add/1 -> Out1/1
  In1/1 -> Demux/1

== system nonlinear_closed_backstepping_0/CRB+CA/Subsystem/skew-symmetric ==
  In1 : Inport
  -x : Fcn  Expr=-1*u[1]
  -y : Fcn  Expr=-1*u[2]
  -z : Fcn  Expr=-1*u[3]
  Constant1 : Constant  Value=0
  Constant2 : Constant  Value=0
  Constant3 : Constant  Value=0
  Matrix Concatenate4 : Concatenate  NumInputs=3  Mode=Multidimensional array  ConcatenateDimension=2
  Matrix Concatenate5 : Concatenate  NumInputs=3  Mode=Multidimensional array  ConcatenateDimension=2
  Matrix Concatenate6 : Concatenate  NumInputs=3  Mode=Multidimensional array  ConcatenateDimension=2
  Matrix Concatenate7 : Concatenate  NumInputs=3  Mode=Multidimensional array
  x : Fcn  Expr=u[1]
  y : Fcn  Expr=u[2]
  z : Fcn  Expr=u[3]
  Out1 : Outport
  wires:
  z/1 -> Matrix Concatenate5/1
  -y/1 -> Matrix Concatenate6/1
  -x/1 -> Matrix Concatenate5/3
  Matrix Concatenate6/1 -> Matrix Concatenate7/3
  Matrix Concatenate4/1 -> Matrix Concatenate7/1
  x/1 -> Matrix Concatenate6/2
  Constant1/1 -> Matrix Concatenate4/1
  -z/1 -> Matrix Concatenate4/2
  y/1 -> Matrix Concatenate4/3
  Constant3/1 -> Matrix Concatenate6/3
  Constant2/1 -> Matrix Concatenate5/2
  Matrix Concatenate5/1 -> Matrix Concatenate7/2
  In1/1 -> -z/1, y/1, z/1, x/1, -y/1, -x/1
  Matrix Concatenate7/1 -> Out1/1

== system nonlinear_closed_backstepping_0/CRB+CA/Subsystem/skew-symmetric1 ==
  In1 : Inport
  -x : Fcn  Expr=-1*u[1]
  -y : Fcn  Expr=-1*u[2]
  -z : Fcn  Expr=-1*u[3]
  Constant1 : Constant  Value=0
  Constant2 : Constant  Value=0
  Constant3 : Constant  Value=0
  Matrix Concatenate4 : Concatenate  NumInputs=3  Mode=Multidimensional array  ConcatenateDimension=2
  Matrix Concatenate5 : Concatenate  NumInputs=3  Mode=Multidimensional array  ConcatenateDimension=2
  Matrix Concatenate6 : Concatenate  NumInputs=3  Mode=Multidimensional array  ConcatenateDimension=2
  Matrix Concatenate7 : Concatenate  NumInputs=3  Mode=Multidimensional array
  x : Fcn  Expr=u[1]
  y : Fcn  Expr=u[2]
  z : Fcn  Expr=u[3]
  Out1 : Outport
  wires:
  z/1 -> Matrix Concatenate5/1
  -y/1 -> Matrix Concatenate6/1
  -x/1 -> Matrix Concatenate5/3
  Matrix Concatenate6/1 -> Matrix Concatenate7/3
  Matrix Concatenate4/1 -> Matrix Concatenate7/1
  x/1 -> Matrix Concatenate6/2
  Constant1/1 -> Matrix Concatenate4/1
  -z/1 -> Matrix Concatenate4/2
  y/1 -> Matrix Concatenate4/3
  Constant3/1 -> Matrix Concatenate6/3
  Constant2/1 -> Matrix Concatenate5/2
  Matrix Concatenate5/1 -> Matrix Concatenate7/2
  In1/1 -> -z/1, y/1, z/1, x/1, -y/1, -x/1
  Matrix Concatenate7/1 -> Out1/1

== system nonlinear_closed_backstepping_0/CRB+CA/Subsystem/skew-symmetric2 ==
  In1 : Inport
  -x : Fcn  Expr=-1*u[1]
  -y : Fcn  Expr=-1*u[2]
  -z : Fcn  Expr=-1*u[3]
  Constant1 : Constant  Value=0
  Constant2 : Constant  Value=0
  Constant3 : Constant  Value=0
  Matrix Concatenate4 : Concatenate  NumInputs=3  Mode=Multidimensional array  ConcatenateDimension=2
  Matrix Concatenate5 : Concatenate  NumInputs=3  Mode=Multidimensional array  ConcatenateDimension=2
  Matrix Concatenate6 : Concatenate  NumInputs=3  Mode=Multidimensional array  ConcatenateDimension=2
  Matrix Concatenate7 : Concatenate  NumInputs=3  Mode=Multidimensional array
  x : Fcn  Expr=u[1]
  y : Fcn  Expr=u[2]
  z : Fcn  Expr=u[3]
  Out1 : Outport
  wires:
  z/1 -> Matrix Concatenate5/1
  -y/1 -> Matrix Concatenate6/1
  -x/1 -> Matrix Concatenate5/3
  Matrix Concatenate6/1 -> Matrix Concatenate7/3
  Matrix Concatenate4/1 -> Matrix Concatenate7/1
  x/1 -> Matrix Concatenate6/2
  Constant1/1 -> Matrix Concatenate4/1
  -z/1 -> Matrix Concatenate4/2
  y/1 -> Matrix Concatenate4/3
  Constant3/1 -> Matrix Concatenate6/3
  Constant2/1 -> Matrix Concatenate5/2
  Matrix Concatenate5/1 -> Matrix Concatenate7/2
  In1/1 -> -z/1, y/1, z/1, x/1, -y/1, -x/1
  Matrix Concatenate7/1 -> Out1/1

== system nonlinear_closed_backstepping_0/CRB+CA/Subsystem/skew-symmetric3 ==
  In1 : Inport
  -x : Fcn  Expr=-1*u[1]
  -y : Fcn  Expr=-1*u[2]
  -z : Fcn  Expr=-1*u[3]
  Constant1 : Constant  Value=0
  Constant2 : Constant  Value=0
  Constant3 : Constant  Value=0
  Matrix Concatenate4 : Concatenate  NumInputs=3  Mode=Multidimensional array  ConcatenateDimension=2
  Matrix Concatenate5 : Concatenate  NumInputs=3  Mode=Multidimensional array  ConcatenateDimension=2
  Matrix Concatenate6 : Concatenate  NumInputs=3  Mode=Multidimensional array  ConcatenateDimension=2
  Matrix Concatenate7 : Concatenate  NumInputs=3  Mode=Multidimensional array
  x : Fcn  Expr=u[1]
  y : Fcn  Expr=u[2]
  z : Fcn  Expr=u[3]
  Out1 : Outport
  wires:
  z/1 -> Matrix Concatenate5/1
  -y/1 -> Matrix Concatenate6/1
  -x/1 -> Matrix Concatenate5/3
  Matrix Concatenate6/1 -> Matrix Concatenate7/3
  Matrix Concatenate4/1 -> Matrix Concatenate7/1
  x/1 -> Matrix Concatenate6/2
  Constant1/1 -> Matrix Concatenate4/1
  -z/1 -> Matrix Concatenate4/2
  y/1 -> Matrix Concatenate4/3
  Constant3/1 -> Matrix Concatenate6/3
  Constant2/1 -> Matrix Concatenate5/2
  Matrix Concatenate5/1 -> Matrix Concatenate7/2
  In1/1 -> -z/1, y/1, z/1, x/1, -y/1, -x/1
  Matrix Concatenate7/1 -> Out1/1

== system nonlinear_closed_backstepping_0/Euler Transformation1/Subsystem4/Dot Product1 ==
